simulink model "ESSSimulation_LFP"  (R2025a)
settings: Solver=VariableStepAuto  StartTime=0.0  StopTime=1800  RelTol=1e-3
undefined symbols (not defined in the file or in its folder): battery_builder_rtmsupport, gcbh
libraries: ANR26650_108S57P_Library_lib x12, fl_lib x4, nesl_utility x4, simulink x1, SignalEditorBlockLib x1
(part 2 of 2)

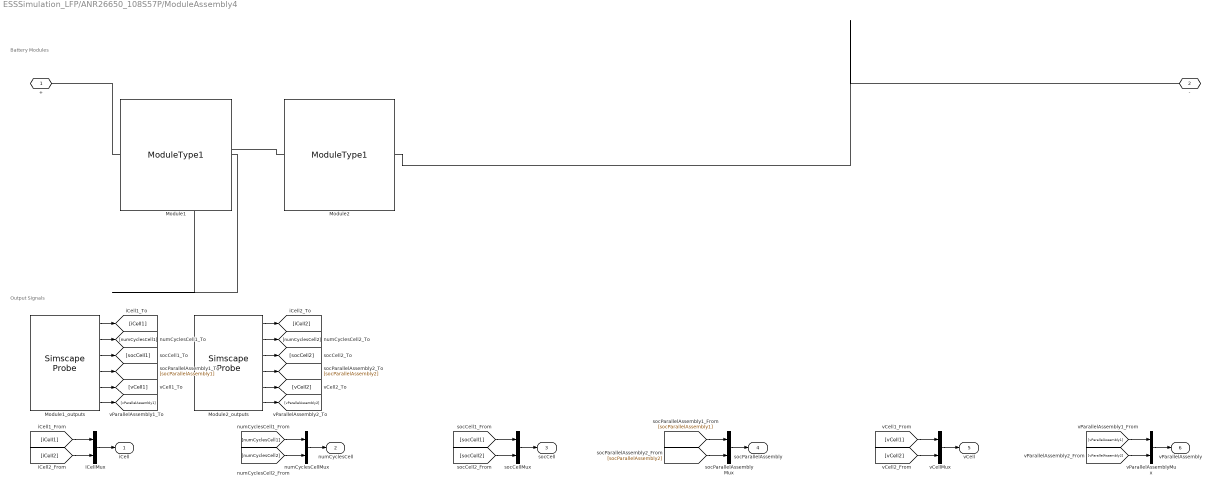
== system ESSSimulation_LFP/ANR26650_108S57P/ModuleAssembly4 ==
  note: Battery Modules
  note: Output Signals
  Module1 : ANR26650_108S57P_Library_lib/Modules/ModuleType1  SOC_vecCell=[0 0.01 0.02 0.03 0.04 0.05 0.06 0.07 0.08 0.09 0.1 0.11 0.12 0.13 0.14 0.15 0.16 0.17 0.18 0.19 0.2 0.21 0.22 0.23 0.24 0.25 0.26 0.27 0.28 0.29 0.3 0.31 0.32 0.33 0.34 0.35 0.36 0.37 0.38 0.39 0.4 0.41 0.42 0.43 0.44 0.45 0.46 0.47 0.48 0.49 0.5 0.51 0.52 0.53 0.54 0.55 0.56 0.57 0.58 0.59 0.6 0.61 0.62 0.63 0.64 0.65 0.66 0.67 0.68 0.69 0.7 0.71 0.72 0.73 0.74 0.75 0.76 0.77 0.78 0.79 0.8 0.81 0.82 0.83 0.84 0.85 0.86 0.87 0.88 0.89 0.9 0.91 0.92 0.93 0.94 0.95 0.96 0.97 0.98 0.99 1]  V0_vecCell=[2.06518 2.68276 2.83127 2.93006 3.00018 3.05444 3.098 3.13677 3.17233 3.19687 3.20429 3.20797 3.21084 3.21322 3.21517 3.22057 3.22301 3.22946 3.23827 3.24173 3.24488 3.24931 3.2535 3.25765 3.26117 3.26357 3.26578 3.26981 3.27407 3.27754 3.27963 3.28165 3.28353 3.28542 3.28715 3.28889 3.29062 3.29275 3.29575 3.29889 3.30203 3.3027 3.30283 3.30242 3.30201 3.30226 3.30369 3.30511 3.3066 3.30845 3.30961 3.31045 3.31128 3.31212 3.31294 3.31336 3.31432 3.31596 3.3176 3.31906 3.32016 3.32147 3.32313 3.32479 3.32699 3.32924 3.33149 3.33281 3.33327 3.33363 3.33398 3.33434 3.33558 3.33748 3.33946 3.34145 3.34404 3.34672 3.34941 3.35026 3.35086 3.35091 3.35083 3.35192 3.35429 3.3566 3.35958 3.36218 3.36335 3.36552 3.36994 3.3722 3.3731 3.37515 3.37949 3.38971 3.40199 3.42645 3.48039 3.63268 3.84587] V  V_rangeCell=[1.8 Inf] V  R0_vecCell=[0.03594 0.04836 0.04765 0.04556 0.04266 0.03932 0.03569 0.03191 0.02805 0.02388 0.02036 0.01833 0.01708 0.01587 0.01474 0.01411 0.01378 0.01359 0.01333 0.01312 0.01302 0.01308 0.01313 0.01318 0.01323 0.01327 0.01333 0.01346 0.0136 0.01363 0.01363 0.01362 0.01361 0.01363 0.01368 0.01374 0.01379 0.01385 0.01395 0.01407 0.01419 0.01424 0.01428 0.01426 0.01424 0.01424 0.01427 0.01431 0.01435 0.01443 0.0145 0.01456 0.01462 0.01468 0.01473 0.01474 0.01476 0.0148 0.01484 0.01488 0.0149 0.01492 0.01498 0.01504 0.01513 0.01523 0.01532 0.01539 0.01543 0.01545 0.01547 0.0155 0.01554 0.01561 0.01566 0.01572 0.0158 0.01589 0.01598 0.01601 0.01605 0.01609 0.01612 0.01613 0.01616 0.01619 0.01618 0.01594 0.0156 0.01534 0.01512 0.01474 0.01431 0.01395 0.01345 0.01301 0.01263 0.01235 0.01272 0.01483 0.01454] Ohm  AHCell=2.341 hr*A  extrapolation_optionCell=simscape.enum.extrapolation.nearest  P=57  S=9  iCell_specify=off  iCell_priority=None  iCell=0 A  iCell_nominal_specify=off  iCell_nominal_value=1  iCell_nominal_unit=A  vCell_specify=off  vCell_priority=None  vCell=0 V  vCell_nominal_specify=off  vCell_nominal_value=1  vCell_nominal_unit=V  socCell_specify=off  socCell_priority=High  socCell=1  socCell_nominal_specify=off  socCell_nominal_value=1  socCell_nominal_unit=1  numCyclesCell_specify=off  numCyclesCell_priority=High  numCyclesCell=0  numCyclesCell_nominal_specify=off  numCyclesCell_nominal_value=1  numCyclesCell_nominal_unit=1  vParallelAssembly_specify=off  vParallelAssembly_priority=None  vParallelAssembly=repmat(0, 9, 1) V  vParallelAssembly_nominal_specify=off  vParallelAssembly_nominal_value=1  vParallelAssembly_nominal_unit=V  socParallelAssembly_specify=off  socParallelAssembly_priority=None  socParallelAssembly=repmat(1, 9, 1)  socParallelAssembly_nominal_specify=off  socParallelAssembly_nominal_value=1  socParallelAssembly_nominal_unit=1
      settings: InternalSimscapePortConfiguration="{\"Bottom\":[{\"id\":\"n\",\"label\":\"-\",\"type\":\"foundation.electrical.electrical\"}],\"Left\":[],\"Right\":[],\"Top\":[{\"id\":\"p\",\"label\":\"+\",\"type\":\"foundation.electrical.electrical\"}]}"
  Module1_outputs : SimscapeProbe  BoundBlock=1095  Variables="{\"iCell\":{\"Probing\":\"ON\"},\"numCyclesCell\":{\"Probing\":\"ON\"},\"socCell\":{\"Probing\":\"ON\"},\"socParallelAssembly\":{\"Probing\":\"ON\"},\"vCell\":{\"Probing\":\"ON\"},\"vParallelAssembly\":{\"Probing\":\"ON\"}}"
  Module2 : ANR26650_108S57P_Library_lib/Modules/ModuleType1  SOC_vecCell=[0 0.01 0.02 0.03 0.04 0.05 0.06 0.07 0.08 0.09 0.1 0.11 0.12 0.13 0.14 0.15 0.16 0.17 0.18 0.19 0.2 0.21 0.22 0.23 0.24 0.25 0.26 0.27 0.28 0.29 0.3 0.31 0.32 0.33 0.34 0.35 0.36 0.37 0.38 0.39 0.4 0.41 0.42 0.43 0.44 0.45 0.46 0.47 0.48 0.49 0.5 0.51 0.52 0.53 0.54 0.55 0.56 0.57 0.58 0.59 0.6 0.61 0.62 0.63 0.64 0.65 0.66 0.67 0.68 0.69 0.7 0.71 0.72 0.73 0.74 0.75 0.76 0.77 0.78 0.79 0.8 0.81 0.82 0.83 0.84 0.85 0.86 0.87 0.88 0.89 0.9 0.91 0.92 0.93 0.94 0.95 0.96 0.97 0.98 0.99 1]  V0_vecCell=[2.06518 2.68276 2.83127 2.93006 3.00018 3.05444 3.098 3.13677 3.17233 3.19687 3.20429 3.20797 3.21084 3.21322 3.21517 3.22057 3.22301 3.22946 3.23827 3.24173 3.24488 3.24931 3.2535 3.25765 3.26117 3.26357 3.26578 3.26981 3.27407 3.27754 3.27963 3.28165 3.28353 3.28542 3.28715 3.28889 3.29062 3.29275 3.29575 3.29889 3.30203 3.3027 3.30283 3.30242 3.30201 3.30226 3.30369 3.30511 3.3066 3.30845 3.30961 3.31045 3.31128 3.31212 3.31294 3.31336 3.31432 3.31596 3.3176 3.31906 3.32016 3.32147 3.32313 3.32479 3.32699 3.32924 3.33149 3.33281 3.33327 3.33363 3.33398 3.33434 3.33558 3.33748 3.33946 3.34145 3.34404 3.34672 3.34941 3.35026 3.35086 3.35091 3.35083 3.35192 3.35429 3.3566 3.35958 3.36218 3.36335 3.36552 3.36994 3.3722 3.3731 3.37515 3.37949 3.38971 3.40199 3.42645 3.48039 3.63268 3.84587] V  V_rangeCell=[1.8 Inf] V  R0_vecCell=[0.03594 0.04836 0.04765 0.04556 0.04266 0.03932 0.03569 0.03191 0.02805 0.02388 0.02036 0.01833 0.01708 0.01587 0.01474 0.01411 0.01378 0.01359 0.01333 0.01312 0.01302 0.01308 0.01313 0.01318 0.01323 0.01327 0.01333 0.01346 0.0136 0.01363 0.01363 0.01362 0.01361 0.01363 0.01368 0.01374 0.01379 0.01385 0.01395 0.01407 0.01419 0.01424 0.01428 0.01426 0.01424 0.01424 0.01427 0.01431 0.01435 0.01443 0.0145 0.01456 0.01462 0.01468 0.01473 0.01474 0.01476 0.0148 0.01484 0.01488 0.0149 0.01492 0.01498 0.01504 0.01513 0.01523 0.01532 0.01539 0.01543 0.01545 0.01547 0.0155 0.01554 0.01561 0.01566 0.01572 0.0158 0.01589 0.01598 0.01601 0.01605 0.01609 0.01612 0.01613 0.01616 0.01619 0.01618 0.01594 0.0156 0.01534 0.01512 0.01474 0.01431 0.01395 0.01345 0.01301 0.01263 0.01235 0.01272 0.01483 0.01454] Ohm  AHCell=2.341 hr*A  extrapolation_optionCell=simscape.enum.extrapolation.nearest  P=57  S=9  iCell_specify=off  iCell_priority=None  iCell=0 A  iCell_nominal_specify=off  iCell_nominal_value=1  iCell_nominal_unit=A  vCell_specify=off  vCell_priority=None  vCell=0 V  vCell_nominal_specify=off  vCell_nominal_value=1  vCell_nominal_unit=V  socCell_specify=off  socCell_priority=High  socCell=1  socCell_nominal_specify=off  socCell_nominal_value=1  socCell_nominal_unit=1  numCyclesCell_specify=off  numCyclesCell_priority=High  numCyclesCell=0  numCyclesCell_nominal_specify=off  numCyclesCell_nominal_value=1  numCyclesCell_nominal_unit=1  vParallelAssembly_specify=off  vParallelAssembly_priority=None  vParallelAssembly=repmat(0, 9, 1) V  vParallelAssembly_nominal_specify=off  vParallelAssembly_nominal_value=1  vParallelAssembly_nominal_unit=V  socParallelAssembly_specify=off  socParallelAssembly_priority=None  socParallelAssembly=repmat(1, 9, 1)  socParallelAssembly_nominal_specify=off  socParallelAssembly_nominal_value=1  socParallelAssembly_nominal_unit=1
      settings: InternalSimscapePortConfiguration="{\"Bottom\":[{\"id\":\"n\",\"label\":\"-\",\"type\":\"foundation.electrical.electrical\"}],\"Left\":[],\"Right\":[],\"Top\":[{\"id\":\"p\",\"label\":\"+\",\"type\":\"foundation.electrical.electrical\"}]}"
  Module2_outputs : SimscapeProbe  BoundBlock=1097  Variables="{\"iCell\":{\"Probing\":\"ON\"},\"numCyclesCell\":{\"Probing\":\"ON\"},\"socCell\":{\"Probing\":\"ON\"},\"socParallelAssembly\":{\"Probing\":\"ON\"},\"vCell\":{\"Probing\":\"ON\"},\"vParallelAssembly\":{\"Probing\":\"ON\"}}"
  iCellMux : Mux  Inputs=2
  numCyclesCellMux : Mux  Inputs=2
  socCellMux : Mux  Inputs=2
  socParallelAssemblyMux : Mux  Inputs=2
  vCellMux : Mux  Inputs=2
  vParallelAssemblyMux : Mux  Inputs=2
  + : PMIOPort  Side=Left
  - : PMIOPort  Port=2  Side=Right
  iCell : Outport
  numCyclesCell : Outport  Port=2
  socCell : Outport  Port=3
  socParallelAssembly : Outport  Port=4
  vCell : Outport  Port=5
  vParallelAssembly : Outport  Port=6
  wires:
  Module1_outputs/1 -> [iCell1]
  iCellMux/1 -> iCell/1
  [iCell1] -> iCellMux/1
  Module1_outputs/2 -> [numCyclesCell1]
  numCyclesCellMux/1 -> numCyclesCell/1
  [numCyclesCell1] -> numCyclesCellMux/1
  Module1_outputs/3 -> [socCell1]
  socCellMux/1 -> socCell/1
  [socCell1] -> socCellMux/1
  Module1_outputs/4 -> [socParallelAssembly1]
  socParallelAssemblyMux/1 -> socParallelAssembly/1
  [socParallelAssembly1] -> socParallelAssemblyMux/1
  Module1_outputs/5 -> [vCell1]
  vCellMux/1 -> vCell/1
  [vCell1] -> vCellMux/1
  Module1_outputs/6 -> [vParallelAssembly1]
  vParallelAssemblyMux/1 -> vParallelAssembly/1
  [vParallelAssembly1] -> vParallelAssemblyMux/1
  Module2_outputs/1 -> [iCell2]
  [iCell2] -> iCellMux/2
  Module2_outputs/2 -> [numCyclesCell2]
  [numCyclesCell2] -> numCyclesCellMux/2
  Module2_outputs/3 -> [socCell2]
  [socCell2] -> socCellMux/2
  Module2_outputs/4 -> [socParallelAssembly2]
  [socParallelAssembly2] -> socParallelAssemblyMux/2
  Module2_outputs/5 -> [vCell2]
  [vCell2] -> vCellMux/2
  Module2_outputs/6 -> [vParallelAssembly2]
  [vParallelAssembly2] -> vParallelAssemblyMux/2
  connections:
  Module2/LConn1 -- Module1/RConn1
  Module1/LConn1 -- +/RConn1
  Module2/RConn1 -- -/RConn1

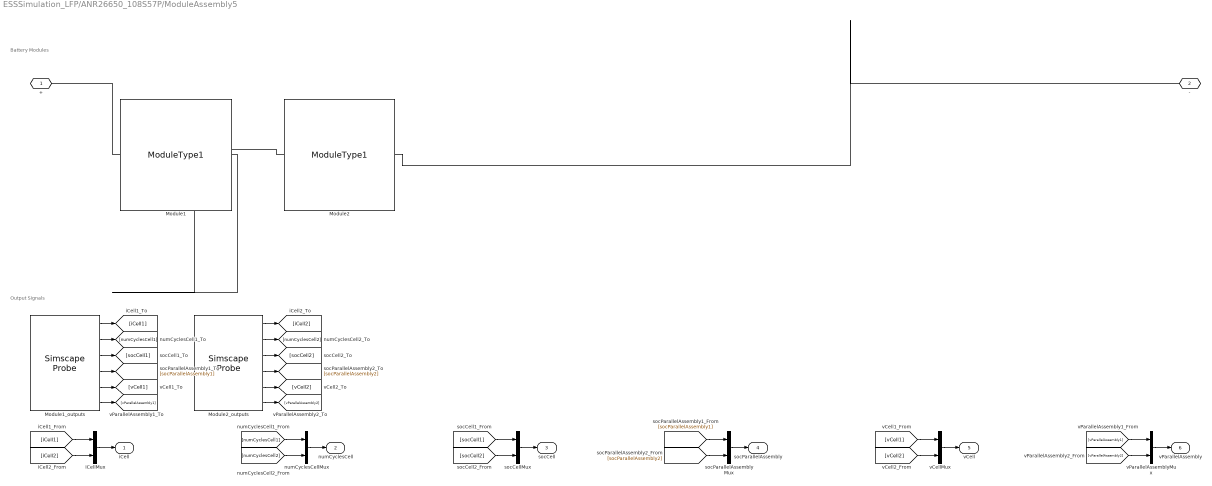
== system ESSSimulation_LFP/ANR26650_108S57P/ModuleAssembly5 ==
  note: Battery Modules
  note: Output Signals
  Module1 : ANR26650_108S57P_Library_lib/Modules/ModuleType1  SOC_vecCell=[0 0.01 0.02 0.03 0.04 0.05 0.06 0.07 0.08 0.09 0.1 0.11 0.12 0.13 0.14 0.15 0.16 0.17 0.18 0.19 0.2 0.21 0.22 0.23 0.24 0.25 0.26 0.27 0.28 0.29 0.3 0.31 0.32 0.33 0.34 0.35 0.36 0.37 0.38 0.39 0.4 0.41 0.42 0.43 0.44 0.45 0.46 0.47 0.48 0.49 0.5 0.51 0.52 0.53 0.54 0.55 0.56 0.57 0.58 0.59 0.6 0.61 0.62 0.63 0.64 0.65 0.66 0.67 0.68 0.69 0.7 0.71 0.72 0.73 0.74 0.75 0.76 0.77 0.78 0.79 0.8 0.81 0.82 0.83 0.84 0.85 0.86 0.87 0.88 0.89 0.9 0.91 0.92 0.93 0.94 0.95 0.96 0.97 0.98 0.99 1]  V0_vecCell=[2.06518 2.68276 2.83127 2.93006 3.00018 3.05444 3.098 3.13677 3.17233 3.19687 3.20429 3.20797 3.21084 3.21322 3.21517 3.22057 3.22301 3.22946 3.23827 3.24173 3.24488 3.24931 3.2535 3.25765 3.26117 3.26357 3.26578 3.26981 3.27407 3.27754 3.27963 3.28165 3.28353 3.28542 3.28715 3.28889 3.29062 3.29275 3.29575 3.29889 3.30203 3.3027 3.30283 3.30242 3.30201 3.30226 3.30369 3.30511 3.3066 3.30845 3.30961 3.31045 3.31128 3.31212 3.31294 3.31336 3.31432 3.31596 3.3176 3.31906 3.32016 3.32147 3.32313 3.32479 3.32699 3.32924 3.33149 3.33281 3.33327 3.33363 3.33398 3.33434 3.33558 3.33748 3.33946 3.34145 3.34404 3.34672 3.34941 3.35026 3.35086 3.35091 3.35083 3.35192 3.35429 3.3566 3.35958 3.36218 3.36335 3.36552 3.36994 3.3722 3.3731 3.37515 3.37949 3.38971 3.40199 3.42645 3.48039 3.63268 3.84587] V  V_rangeCell=[1.8 Inf] V  R0_vecCell=[0.03594 0.04836 0.04765 0.04556 0.04266 0.03932 0.03569 0.03191 0.02805 0.02388 0.02036 0.01833 0.01708 0.01587 0.01474 0.01411 0.01378 0.01359 0.01333 0.01312 0.01302 0.01308 0.01313 0.01318 0.01323 0.01327 0.01333 0.01346 0.0136 0.01363 0.01363 0.01362 0.01361 0.01363 0.01368 0.01374 0.01379 0.01385 0.01395 0.01407 0.01419 0.01424 0.01428 0.01426 0.01424 0.01424 0.01427 0.01431 0.01435 0.01443 0.0145 0.01456 0.01462 0.01468 0.01473 0.01474 0.01476 0.0148 0.01484 0.01488 0.0149 0.01492 0.01498 0.01504 0.01513 0.01523 0.01532 0.01539 0.01543 0.01545 0.01547 0.0155 0.01554 0.01561 0.01566 0.01572 0.0158 0.01589 0.01598 0.01601 0.01605 0.01609 0.01612 0.01613 0.01616 0.01619 0.01618 0.01594 0.0156 0.01534 0.01512 0.01474 0.01431 0.01395 0.01345 0.01301 0.01263 0.01235 0.01272 0.01483 0.01454] Ohm  AHCell=2.341 hr*A  extrapolation_optionCell=simscape.enum.extrapolation.nearest  P=57  S=9  iCell_specify=off  iCell_priority=None  iCell=0 A  iCell_nominal_specify=off  iCell_nominal_value=1  iCell_nominal_unit=A  vCell_specify=off  vCell_priority=None  vCell=0 V  vCell_nominal_specify=off  vCell_nominal_value=1  vCell_nominal_unit=V  socCell_specify=off  socCell_priority=High  socCell=1  socCell_nominal_specify=off  socCell_nominal_value=1  socCell_nominal_unit=1  numCyclesCell_specify=off  numCyclesCell_priority=High  numCyclesCell=0  numCyclesCell_nominal_specify=off  numCyclesCell_nominal_value=1  numCyclesCell_nominal_unit=1  vParallelAssembly_specify=off  vParallelAssembly_priority=None  vParallelAssembly=repmat(0, 9, 1) V  vParallelAssembly_nominal_specify=off  vParallelAssembly_nominal_value=1  vParallelAssembly_nominal_unit=V  socParallelAssembly_specify=off  socParallelAssembly_priority=None  socParallelAssembly=repmat(1, 9, 1)  socParallelAssembly_nominal_specify=off  socParallelAssembly_nominal_value=1  socParallelAssembly_nominal_unit=1
      settings: InternalSimscapePortConfiguration="{\"Bottom\":[{\"id\":\"n\",\"label\":\"-\",\"type\":\"foundation.electrical.electrical\"}],\"Left\":[],\"Right\":[],\"Top\":[{\"id\":\"p\",\"label\":\"+\",\"type\":\"foundation.electrical.electrical\"}]}"
  Module1_outputs : SimscapeProbe  BoundBlock=1140  Variables="{\"iCell\":{\"Probing\":\"ON\"},\"numCyclesCell\":{\"Probing\":\"ON\"},\"socCell\":{\"Probing\":\"ON\"},\"socParallelAssembly\":{\"Probing\":\"ON\"},\"vCell\":{\"Probing\":\"ON\"},\"vParallelAssembly\":{\"Probing\":\"ON\"}}"
  Module2 : ANR26650_108S57P_Library_lib/Modules/ModuleType1  SOC_vecCell=[0 0.01 0.02 0.03 0.04 0.05 0.06 0.07 0.08 0.09 0.1 0.11 0.12 0.13 0.14 0.15 0.16 0.17 0.18 0.19 0.2 0.21 0.22 0.23 0.24 0.25 0.26 0.27 0.28 0.29 0.3 0.31 0.32 0.33 0.34 0.35 0.36 0.37 0.38 0.39 0.4 0.41 0.42 0.43 0.44 0.45 0.46 0.47 0.48 0.49 0.5 0.51 0.52 0.53 0.54 0.55 0.56 0.57 0.58 0.59 0.6 0.61 0.62 0.63 0.64 0.65 0.66 0.67 0.68 0.69 0.7 0.71 0.72 0.73 0.74 0.75 0.76 0.77 0.78 0.79 0.8 0.81 0.82 0.83 0.84 0.85 0.86 0.87 0.88 0.89 0.9 0.91 0.92 0.93 0.94 0.95 0.96 0.97 0.98 0.99 1]  V0_vecCell=[2.06518 2.68276 2.83127 2.93006 3.00018 3.05444 3.098 3.13677 3.17233 3.19687 3.20429 3.20797 3.21084 3.21322 3.21517 3.22057 3.22301 3.22946 3.23827 3.24173 3.24488 3.24931 3.2535 3.25765 3.26117 3.26357 3.26578 3.26981 3.27407 3.27754 3.27963 3.28165 3.28353 3.28542 3.28715 3.28889 3.29062 3.29275 3.29575 3.29889 3.30203 3.3027 3.30283 3.30242 3.30201 3.30226 3.30369 3.30511 3.3066 3.30845 3.30961 3.31045 3.31128 3.31212 3.31294 3.31336 3.31432 3.31596 3.3176 3.31906 3.32016 3.32147 3.32313 3.32479 3.32699 3.32924 3.33149 3.33281 3.33327 3.33363 3.33398 3.33434 3.33558 3.33748 3.33946 3.34145 3.34404 3.34672 3.34941 3.35026 3.35086 3.35091 3.35083 3.35192 3.35429 3.3566 3.35958 3.36218 3.36335 3.36552 3.36994 3.3722 3.3731 3.37515 3.37949 3.38971 3.40199 3.42645 3.48039 3.63268 3.84587] V  V_rangeCell=[1.8 Inf] V  R0_vecCell=[0.03594 0.04836 0.04765 0.04556 0.04266 0.03932 0.03569 0.03191 0.02805 0.02388 0.02036 0.01833 0.01708 0.01587 0.01474 0.01411 0.01378 0.01359 0.01333 0.01312 0.01302 0.01308 0.01313 0.01318 0.01323 0.01327 0.01333 0.01346 0.0136 0.01363 0.01363 0.01362 0.01361 0.01363 0.01368 0.01374 0.01379 0.01385 0.01395 0.01407 0.01419 0.01424 0.01428 0.01426 0.01424 0.01424 0.01427 0.01431 0.01435 0.01443 0.0145 0.01456 0.01462 0.01468 0.01473 0.01474 0.01476 0.0148 0.01484 0.01488 0.0149 0.01492 0.01498 0.01504 0.01513 0.01523 0.01532 0.01539 0.01543 0.01545 0.01547 0.0155 0.01554 0.01561 0.01566 0.01572 0.0158 0.01589 0.01598 0.01601 0.01605 0.01609 0.01612 0.01613 0.01616 0.01619 0.01618 0.01594 0.0156 0.01534 0.01512 0.01474 0.01431 0.01395 0.01345 0.01301 0.01263 0.01235 0.01272 0.01483 0.01454] Ohm  AHCell=2.341 hr*A  extrapolation_optionCell=simscape.enum.extrapolation.nearest  P=57  S=9  iCell_specify=off  iCell_priority=None  iCell=0 A  iCell_nominal_specify=off  iCell_nominal_value=1  iCell_nominal_unit=A  vCell_specify=off  vCell_priority=None  vCell=0 V  vCell_nominal_specify=off  vCell_nominal_value=1  vCell_nominal_unit=V  socCell_specify=off  socCell_priority=High  socCell=1  socCell_nominal_specify=off  socCell_nominal_value=1  socCell_nominal_unit=1  numCyclesCell_specify=off  numCyclesCell_priority=High  numCyclesCell=0  numCyclesCell_nominal_specify=off  numCyclesCell_nominal_value=1  numCyclesCell_nominal_unit=1  vParallelAssembly_specify=off  vParallelAssembly_priority=None  vParallelAssembly=repmat(0, 9, 1) V  vParallelAssembly_nominal_specify=off  vParallelAssembly_nominal_value=1  vParallelAssembly_nominal_unit=V  socParallelAssembly_specify=off  socParallelAssembly_priority=None  socParallelAssembly=repmat(1, 9, 1)  socParallelAssembly_nominal_specify=off  socParallelAssembly_nominal_value=1  socParallelAssembly_nominal_unit=1
      settings: InternalSimscapePortConfiguration="{\"Bottom\":[{\"id\":\"n\",\"label\":\"-\",\"type\":\"foundation.electrical.electrical\"}],\"Left\":[],\"Right\":[],\"Top\":[{\"id\":\"p\",\"label\":\"+\",\"type\":\"foundation.electrical.electrical\"}]}"
  Module2_outputs : SimscapeProbe  BoundBlock=1142  Variables="{\"iCell\":{\"Probing\":\"ON\"},\"numCyclesCell\":{\"Probing\":\"ON\"},\"socCell\":{\"Probing\":\"ON\"},\"socParallelAssembly\":{\"Probing\":\"ON\"},\"vCell\":{\"Probing\":\"ON\"},\"vParallelAssembly\":{\"Probing\":\"ON\"}}"
  iCellMux : Mux  Inputs=2
  numCyclesCellMux : Mux  Inputs=2
  socCellMux : Mux  Inputs=2
  socParallelAssemblyMux : Mux  Inputs=2
  vCellMux : Mux  Inputs=2
  vParallelAssemblyMux : Mux  Inputs=2
  + : PMIOPort  Side=Left
  - : PMIOPort  Port=2  Side=Right
  iCell : Outport
  numCyclesCell : Outport  Port=2
  socCell : Outport  Port=3
  socParallelAssembly : Outport  Port=4
  vCell : Outport  Port=5
  vParallelAssembly : Outport  Port=6
  wires:
  Module1_outputs/1 -> [iCell1]
  iCellMux/1 -> iCell/1
  [iCell1] -> iCellMux/1
  Module1_outputs/2 -> [numCyclesCell1]
  numCyclesCellMux/1 -> numCyclesCell/1
  [numCyclesCell1] -> numCyclesCellMux/1
  Module1_outputs/3 -> [socCell1]
  socCellMux/1 -> socCell/1
  [socCell1] -> socCellMux/1
  Module1_outputs/4 -> [socParallelAssembly1]
  socParallelAssemblyMux/1 -> socParallelAssembly/1
  [socParallelAssembly1] -> socParallelAssemblyMux/1
  Module1_outputs/5 -> [vCell1]
  vCellMux/1 -> vCell/1
  [vCell1] -> vCellMux/1
  Module1_outputs/6 -> [vParallelAssembly1]
  vParallelAssemblyMux/1 -> vParallelAssembly/1
  [vParallelAssembly1] -> vParallelAssemblyMux/1
  Module2_outputs/1 -> [iCell2]
  [iCell2] -> iCellMux/2
  Module2_outputs/2 -> [numCyclesCell2]
  [numCyclesCell2] -> numCyclesCellMux/2
  Module2_outputs/3 -> [socCell2]
  [socCell2] -> socCellMux/2
  Module2_outputs/4 -> [socParallelAssembly2]
  [socParallelAssembly2] -> socParallelAssemblyMux/2
  Module2_outputs/5 -> [vCell2]
  [vCell2] -> vCellMux/2
  Module2_outputs/6 -> [vParallelAssembly2]
  [vParallelAssembly2] -> vParallelAssemblyMux/2
  connections:
  Module2/LConn1 -- Module1/RConn1
  Module1/LConn1 -- +/RConn1
  Module2/RConn1 -- -/RConn1

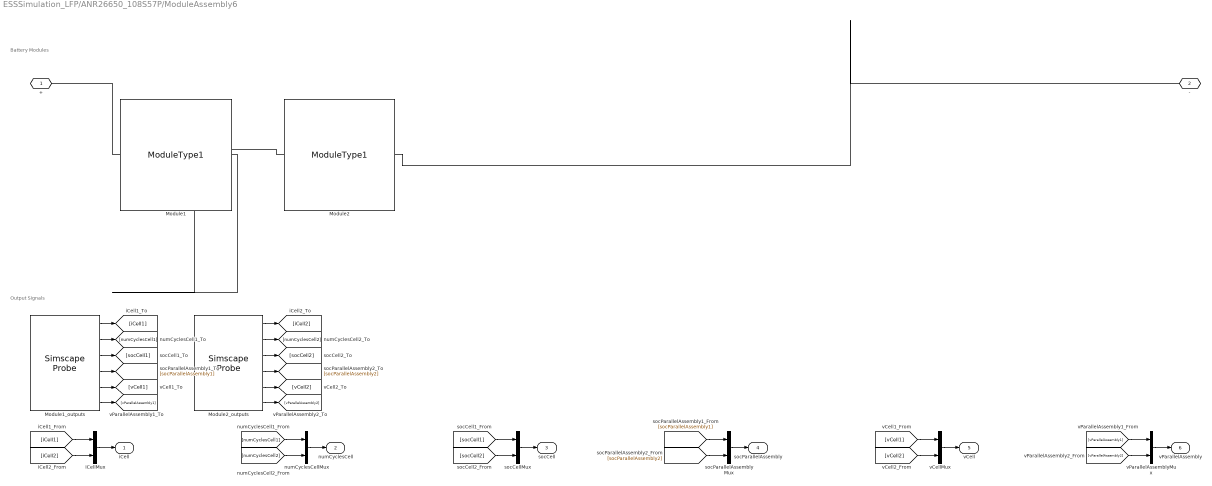
== system ESSSimulation_LFP/ANR26650_108S57P/ModuleAssembly6 ==
  note: Battery Modules
  note: Output Signals
  Module1 : ANR26650_108S57P_Library_lib/Modules/ModuleType1  SOC_vecCell=[0 0.01 0.02 0.03 0.04 0.05 0.06 0.07 0.08 0.09 0.1 0.11 0.12 0.13 0.14 0.15 0.16 0.17 0.18 0.19 0.2 0.21 0.22 0.23 0.24 0.25 0.26 0.27 0.28 0.29 0.3 0.31 0.32 0.33 0.34 0.35 0.36 0.37 0.38 0.39 0.4 0.41 0.42 0.43 0.44 0.45 0.46 0.47 0.48 0.49 0.5 0.51 0.52 0.53 0.54 0.55 0.56 0.57 0.58 0.59 0.6 0.61 0.62 0.63 0.64 0.65 0.66 0.67 0.68 0.69 0.7 0.71 0.72 0.73 0.74 0.75 0.76 0.77 0.78 0.79 0.8 0.81 0.82 0.83 0.84 0.85 0.86 0.87 0.88 0.89 0.9 0.91 0.92 0.93 0.94 0.95 0.96 0.97 0.98 0.99 1]  V0_vecCell=[2.06518 2.68276 2.83127 2.93006 3.00018 3.05444 3.098 3.13677 3.17233 3.19687 3.20429 3.20797 3.21084 3.21322 3.21517 3.22057 3.22301 3.22946 3.23827 3.24173 3.24488 3.24931 3.2535 3.25765 3.26117 3.26357 3.26578 3.26981 3.27407 3.27754 3.27963 3.28165 3.28353 3.28542 3.28715 3.28889 3.29062 3.29275 3.29575 3.29889 3.30203 3.3027 3.30283 3.30242 3.30201 3.30226 3.30369 3.30511 3.3066 3.30845 3.30961 3.31045 3.31128 3.31212 3.31294 3.31336 3.31432 3.31596 3.3176 3.31906 3.32016 3.32147 3.32313 3.32479 3.32699 3.32924 3.33149 3.33281 3.33327 3.33363 3.33398 3.33434 3.33558 3.33748 3.33946 3.34145 3.34404 3.34672 3.34941 3.35026 3.35086 3.35091 3.35083 3.35192 3.35429 3.3566 3.35958 3.36218 3.36335 3.36552 3.36994 3.3722 3.3731 3.37515 3.37949 3.38971 3.40199 3.42645 3.48039 3.63268 3.84587] V  V_rangeCell=[1.8 Inf] V  R0_vecCell=[0.03594 0.04836 0.04765 0.04556 0.04266 0.03932 0.03569 0.03191 0.02805 0.02388 0.02036 0.01833 0.01708 0.01587 0.01474 0.01411 0.01378 0.01359 0.01333 0.01312 0.01302 0.01308 0.01313 0.01318 0.01323 0.01327 0.01333 0.01346 0.0136 0.01363 0.01363 0.01362 0.01361 0.01363 0.01368 0.01374 0.01379 0.01385 0.01395 0.01407 0.01419 0.01424 0.01428 0.01426 0.01424 0.01424 0.01427 0.01431 0.01435 0.01443 0.0145 0.01456 0.01462 0.01468 0.01473 0.01474 0.01476 0.0148 0.01484 0.01488 0.0149 0.01492 0.01498 0.01504 0.01513 0.01523 0.01532 0.01539 0.01543 0.01545 0.01547 0.0155 0.01554 0.01561 0.01566 0.01572 0.0158 0.01589 0.01598 0.01601 0.01605 0.01609 0.01612 0.01613 0.01616 0.01619 0.01618 0.01594 0.0156 0.01534 0.01512 0.01474 0.01431 0.01395 0.01345 0.01301 0.01263 0.01235 0.01272 0.01483 0.01454] Ohm  AHCell=2.341 hr*A  extrapolation_optionCell=simscape.enum.extrapolation.nearest  P=57  S=9  iCell_specify=off  iCell_priority=None  iCell=0 A  iCell_nominal_specify=off  iCell_nominal_value=1  iCell_nominal_unit=A  vCell_specify=off  vCell_priority=None  vCell=0 V  vCell_nominal_specify=off  vCell_nominal_value=1  vCell_nominal_unit=V  socCell_specify=off  socCell_priority=High  socCell=1  socCell_nominal_specify=off  socCell_nominal_value=1  socCell_nominal_unit=1  numCyclesCell_specify=off  numCyclesCell_priority=High  numCyclesCell=0  numCyclesCell_nominal_specify=off  numCyclesCell_nominal_value=1  numCyclesCell_nominal_unit=1  vParallelAssembly_specify=off  vParallelAssembly_priority=None  vParallelAssembly=repmat(0, 9, 1) V  vParallelAssembly_nominal_specify=off  vParallelAssembly_nominal_value=1  vParallelAssembly_nominal_unit=V  socParallelAssembly_specify=off  socParallelAssembly_priority=None  socParallelAssembly=repmat(1, 9, 1)  socParallelAssembly_nominal_specify=off  socParallelAssembly_nominal_value=1  socParallelAssembly_nominal_unit=1
      settings: InternalSimscapePortConfiguration="{\"Bottom\":[{\"id\":\"n\",\"label\":\"-\",\"type\":\"foundation.electrical.electrical\"}],\"Left\":[],\"Right\":[],\"Top\":[{\"id\":\"p\",\"label\":\"+\",\"type\":\"foundation.electrical.electrical\"}]}"
  Module1_outputs : SimscapeProbe  BoundBlock=1185  Variables="{\"iCell\":{\"Probing\":\"ON\"},\"numCyclesCell\":{\"Probing\":\"ON\"},\"socCell\":{\"Probing\":\"ON\"},\"socParallelAssembly\":{\"Probing\":\"ON\"},\"vCell\":{\"Probing\":\"ON\"},\"vParallelAssembly\":{\"Probing\":\"ON\"}}"
  Module2 : ANR26650_108S57P_Library_lib/Modules/ModuleType1  SOC_vecCell=[0 0.01 0.02 0.03 0.04 0.05 0.06 0.07 0.08 0.09 0.1 0.11 0.12 0.13 0.14 0.15 0.16 0.17 0.18 0.19 0.2 0.21 0.22 0.23 0.24 0.25 0.26 0.27 0.28 0.29 0.3 0.31 0.32 0.33 0.34 0.35 0.36 0.37 0.38 0.39 0.4 0.41 0.42 0.43 0.44 0.45 0.46 0.47 0.48 0.49 0.5 0.51 0.52 0.53 0.54 0.55 0.56 0.57 0.58 0.59 0.6 0.61 0.62 0.63 0.64 0.65 0.66 0.67 0.68 0.69 0.7 0.71 0.72 0.73 0.74 0.75 0.76 0.77 0.78 0.79 0.8 0.81 0.82 0.83 0.84 0.85 0.86 0.87 0.88 0.89 0.9 0.91 0.92 0.93 0.94 0.95 0.96 0.97 0.98 0.99 1]  V0_vecCell=[2.06518 2.68276 2.83127 2.93006 3.00018 3.05444 3.098 3.13677 3.17233 3.19687 3.20429 3.20797 3.21084 3.21322 3.21517 3.22057 3.22301 3.22946 3.23827 3.24173 3.24488 3.24931 3.2535 3.25765 3.26117 3.26357 3.26578 3.26981 3.27407 3.27754 3.27963 3.28165 3.28353 3.28542 3.28715 3.28889 3.29062 3.29275 3.29575 3.29889 3.30203 3.3027 3.30283 3.30242 3.30201 3.30226 3.30369 3.30511 3.3066 3.30845 3.30961 3.31045 3.31128 3.31212 3.31294 3.31336 3.31432 3.31596 3.3176 3.31906 3.32016 3.32147 3.32313 3.32479 3.32699 3.32924 3.33149 3.33281 3.33327 3.33363 3.33398 3.33434 3.33558 3.33748 3.33946 3.34145 3.34404 3.34672 3.34941 3.35026 3.35086 3.35091 3.35083 3.35192 3.35429 3.3566 3.35958 3.36218 3.36335 3.36552 3.36994 3.3722 3.3731 3.37515 3.37949 3.38971 3.40199 3.42645 3.48039 3.63268 3.84587] V  V_rangeCell=[1.8 Inf] V  R0_vecCell=[0.03594 0.04836 0.04765 0.04556 0.04266 0.03932 0.03569 0.03191 0.02805 0.02388 0.02036 0.01833 0.01708 0.01587 0.01474 0.01411 0.01378 0.01359 0.01333 0.01312 0.01302 0.01308 0.01313 0.01318 0.01323 0.01327 0.01333 0.01346 0.0136 0.01363 0.01363 0.01362 0.01361 0.01363 0.01368 0.01374 0.01379 0.01385 0.01395 0.01407 0.01419 0.01424 0.01428 0.01426 0.01424 0.01424 0.01427 0.01431 0.01435 0.01443 0.0145 0.01456 0.01462 0.01468 0.01473 0.01474 0.01476 0.0148 0.01484 0.01488 0.0149 0.01492 0.01498 0.01504 0.01513 0.01523 0.01532 0.01539 0.01543 0.01545 0.01547 0.0155 0.01554 0.01561 0.01566 0.01572 0.0158 0.01589 0.01598 0.01601 0.01605 0.01609 0.01612 0.01613 0.01616 0.01619 0.01618 0.01594 0.0156 0.01534 0.01512 0.01474 0.01431 0.01395 0.01345 0.01301 0.01263 0.01235 0.01272 0.01483 0.01454] Ohm  AHCell=2.341 hr*A  extrapolation_optionCell=simscape.enum.extrapolation.nearest  P=57  S=9  iCell_specify=off  iCell_priority=None  iCell=0 A  iCell_nominal_specify=off  iCell_nominal_value=1  iCell_nominal_unit=A  vCell_specify=off  vCell_priority=None  vCell=0 V  vCell_nominal_specify=off  vCell_nominal_value=1  vCell_nominal_unit=V  socCell_specify=off  socCell_priority=High  socCell=1  socCell_nominal_specify=off  socCell_nominal_value=1  socCell_nominal_unit=1  numCyclesCell_specify=off  numCyclesCell_priority=High  numCyclesCell=0  numCyclesCell_nominal_specify=off  numCyclesCell_nominal_value=1  numCyclesCell_nominal_unit=1  vParallelAssembly_specify=off  vParallelAssembly_priority=None  vParallelAssembly=repmat(0, 9, 1) V  vParallelAssembly_nominal_specify=off  vParallelAssembly_nominal_value=1  vParallelAssembly_nominal_unit=V  socParallelAssembly_specify=off  socParallelAssembly_priority=None  socParallelAssembly=repmat(1, 9, 1)  socParallelAssembly_nominal_specify=off  socParallelAssembly_nominal_value=1  socParallelAssembly_nominal_unit=1
      settings: InternalSimscapePortConfiguration="{\"Bottom\":[{\"id\":\"n\",\"label\":\"-\",\"type\":\"foundation.electrical.electrical\"}],\"Left\":[],\"Right\":[],\"Top\":[{\"id\":\"p\",\"label\":\"+\",\"type\":\"foundation.electrical.electrical\"}]}"
  Module2_outputs : SimscapeProbe  BoundBlock=1187  Variables="{\"iCell\":{\"Probing\":\"ON\"},\"numCyclesCell\":{\"Probing\":\"ON\"},\"socCell\":{\"Probing\":\"ON\"},\"socParallelAssembly\":{\"Probing\":\"ON\"},\"vCell\":{\"Probing\":\"ON\"},\"vParallelAssembly\":{\"Probing\":\"ON\"}}"
  iCellMux : Mux  Inputs=2
  numCyclesCellMux : Mux  Inputs=2
  socCellMux : Mux  Inputs=2
  socParallelAssemblyMux : Mux  Inputs=2
  vCellMux : Mux  Inputs=2
  vParallelAssemblyMux : Mux  Inputs=2
  + : PMIOPort  Side=Left
  - : PMIOPort  Port=2  Side=Right
  iCell : Outport
  numCyclesCell : Outport  Port=2
  socCell : Outport  Port=3
  socParallelAssembly : Outport  Port=4
  vCell : Outport  Port=5
  vParallelAssembly : Outport  Port=6
  wires:
  Module1_outputs/1 -> [iCell1]
  iCellMux/1 -> iCell/1
  [iCell1] -> iCellMux/1
  Module1_outputs/2 -> [numCyclesCell1]
  numCyclesCellMux/1 -> numCyclesCell/1
  [numCyclesCell1] -> numCyclesCellMux/1
  Module1_outputs/3 -> [socCell1]
  socCellMux/1 -> socCell/1
  [socCell1] -> socCellMux/1
  Module1_outputs/4 -> [socParallelAssembly1]
  socParallelAssemblyMux/1 -> socParallelAssembly/1
  [socParallelAssembly1] -> socParallelAssemblyMux/1
  Module1_outputs/5 -> [vCell1]
  vCellMux/1 -> vCell/1
  [vCell1] -> vCellMux/1
  Module1_outputs/6 -> [vParallelAssembly1]
  vParallelAssemblyMux/1 -> vParallelAssembly/1
  [vParallelAssembly1] -> vParallelAssemblyMux/1
  Module2_outputs/1 -> [iCell2]
  [iCell2] -> iCellMux/2
  Module2_outputs/2 -> [numCyclesCell2]
  [numCyclesCell2] -> numCyclesCellMux/2
  Module2_outputs/3 -> [socCell2]
  [socCell2] -> socCellMux/2
  Module2_outputs/4 -> [socParallelAssembly2]
  [socParallelAssembly2] -> socParallelAssemblyMux/2
  Module2_outputs/5 -> [vCell2]
  [vCell2] -> vCellMux/2
  Module2_outputs/6 -> [vParallelAssembly2]
  [vParallelAssembly2] -> vParallelAssemblyMux/2
  connections:
  Module2/LConn1 -- Module1/RConn1
  Module1/LConn1 -- +/RConn1
  Module2/RConn1 -- -/RConn1
